simulink model "QDrone_YOLO_Stage6_RealYOLO_MonitorOnly"  (R2021b)
settings: Solver=ode2  StartTime=0.0  StopTime=inf  FixedStep=0.001  RelTol=1e-3  EnableMultiTasking=on
undefined symbols (not defined in the file): Host, qc_get_step_size
libraries: quarc_library x33, simulink x5
(part 2 of 2)

== system QDrone_YOLO_Stage6_RealYOLO_MonitorOnly/MISSION SERVER - LEADER//FOLLOWER with QBot 2e and QDrone/JOYSTICK/Pulse Check ==
  note: For this subsystem we will count the number of new pulses. The data can be considered enabled once the count of new signals has gone beyond 1. This will enable the Initializing and conditioning subsystem.
  new : Inport
  Compare : quarc_library/Logic Operations/Compare  operator=>=  output_data_type=boolean
      settings: SourceProductName=QUARC Targets
  Pulse Check : Constant
  "pulse count " : Subsystem  TreatAsAtomicUnit=on
  signal enable : Outport  InitialOutput=0  VectorParamsAs1DForOutWhenUnconnected=off
  wires:
  Compare/1 -> signal enable/1
  Pulse Check/1 -> Compare/2
  new/1 -> "pulse count "/Trigger
  "pulse count "/1(Number of Pulses) -> Compare/1

== system QDrone_YOLO_Stage6_RealYOLO_MonitorOnly/MISSION SERVER - LEADER//FOLLOWER with QBot 2e and QDrone/Data Server (Localization) /Convention Correction (Motive Frame to Research Studio Frame) - QBot 2e/Prevent Gimbal Lock ==
  note: Remapping the rotation order to prevent gimbal lock
      | in heading/yaw due to Euler singularity condition
  Attitude (rad) [3] : Inport
  Demux : Demux  Outputs=3
  Euler Angles from Rotation Matrix (Relative ZYX) : quarc_library/Math Operations/Matrices/Euler Angles from Rotation Matrix  menu_order=Relative Z-Y-X
      settings: SourceProductName=QUARC Targets
  Euler Angles to Rotation Matrix (Relative YZX) : quarc_library/Math Operations/Matrices/Euler Angles to Rotation Matrix  menu_order=Relative Y-Z-X
      settings: SourceProductName=QUARC Targets
  Mux : Mux  Inputs=3
  "Attitude (rad) [3] " : Outport  VectorParamsAs1DForOutWhenUnconnected=off
  wires:
  Euler Angles from Rotation Matrix (Relative ZYX)/2 -> Mux/2
  Euler Angles from Rotation Matrix (Relative ZYX)/1 -> Mux/3
  Euler Angles from Rotation Matrix (Relative ZYX)/3 -> Mux/1
  Euler Angles to Rotation Matrix (Relative YZX)/1 -> Euler Angles from Rotation Matrix (Relative ZYX)/1
  Attitude (rad) [3]/1 -> Demux/1
  Mux/1 -> "Attitude (rad) [3] "/1
  Demux/2 -> Euler Angles to Rotation Matrix (Relative YZX)/1
  Demux/3 -> Euler Angles to Rotation Matrix (Relative YZX)/2
  Demux/1 -> Euler Angles to Rotation Matrix (Relative YZX)/3

== system QDrone_YOLO_Stage6_RealYOLO_MonitorOnly/MISSION SERVER - LEADER//FOLLOWER with QBot 2e and QDrone/Data Server (Localization) /Convention Correction (Motive Frame to Research Studio Frame) - QDrone/Prevent Gimbal Lock ==
  note: Remapping the rotation order to prevent gimbal lock
      | in heading/yaw due to Euler singularity condition
  Attitude (rad) [3] : Inport
  Demux : Demux  Outputs=3
  Euler Angles from Rotation Matrix (Relative ZYX) : quarc_library/Math Operations/Matrices/Euler Angles from Rotation Matrix  menu_order=Relative Z-Y-X
      settings: SourceProductName=QUARC Targets
  Euler Angles to Rotation Matrix (Relative YZX) : quarc_library/Math Operations/Matrices/Euler Angles to Rotation Matrix  menu_order=Relative Y-Z-X
      settings: SourceProductName=QUARC Targets
  Mux : Mux  Inputs=3
  "Attitude (rad) [3] " : Outport  VectorParamsAs1DForOutWhenUnconnected=off
  wires:
  Euler Angles from Rotation Matrix (Relative ZYX)/2 -> Mux/2
  Euler Angles from Rotation Matrix (Relative ZYX)/1 -> Mux/3
  Euler Angles from Rotation Matrix (Relative ZYX)/3 -> Mux/1
  Euler Angles to Rotation Matrix (Relative YZX)/1 -> Euler Angles from Rotation Matrix (Relative ZYX)/1
  Attitude (rad) [3]/1 -> Demux/1
  Mux/1 -> "Attitude (rad) [3] "/1
  Demux/2 -> Euler Angles to Rotation Matrix (Relative YZX)/1
  Demux/3 -> Euler Angles to Rotation Matrix (Relative YZX)/2
  Demux/1 -> Euler Angles to Rotation Matrix (Relative YZX)/3

== system QDrone_YOLO_Stage6_RealYOLO_MonitorOnly/MISSION SERVER - LEADER//FOLLOWER with QBot 2e and QDrone/JOYSTICK/Pulse Check/pulse count  ==
  Trigger : TriggerPort  TriggerType=either  VariantControl=Variant
  Constant1 : Constant  Value=0
  Increment Stored Integer : simulink/Additional Math & Discrete/Additional Math: Increment - Decrement/Increment Stored Integer
  Sum : Sum  Inputs=|++
  Unit Delay : UnitDelay  SampleTime=-1  HasFrameUpgradeWarning=on
  Number of Pulses : Outport  VectorParamsAs1DForOutWhenUnconnected=off
  wires:
  Constant1/1 -> Sum/1
  Sum/1 -> Increment Stored Integer/1
  Unit Delay/1 -> Sum/2
  Increment Stored Integer/1 -> Unit Delay/1, Number of Pulses/1

== matlab function QDrone_YOLO_Stage6_RealYOLO_MonitorOnly/MISSION SERVER - LEADER//FOLLOWER with QBot 2e and QDrone/Extract Vehicle Data - QBot 2e/Extract Object Data ==
  data: data input; position output; orientation output; index input; tracking output
function [position, orientation, tracking] = fcn(data, index)

n = length(data)/7;

if (index<=0)||(index>n)
    position = zeros(1,3); orientation = zeros(1,3); tracking = 0;
else
    position = [data(index*3-2), data(index*3-1), data(index*3)];
    orientation = [data((index+n)*3 - 2), data((index+n)*3 - 1), data((index+n)*3)];
    tracking = data(index + (n*6));
end

== matlab function QDrone_YOLO_Stage6_RealYOLO_MonitorOnly/MISSION SERVER - LEADER//FOLLOWER with QBot 2e and QDrone/Extract Vehicle Data - QDrone/Extract Object Data ==
  data: data input; position output; orientation output; index input; tracking output
function [position, orientation, tracking] = fcn(data, index)

n = length(data)/7;

if (index<=0)||(index>n)
    position = zeros(1,3); orientation = zeros(1,3); tracking = 0;
else
    position = [data(index*3-2), data(index*3-1), data(index*3)];
    orientation = [data((index+n)*3 - 2), data((index+n)*3 - 1), data((index+n)*3)];
    tracking = data(index + (n*6));
end

== matlab function QDrone_YOLO_Stage6_RealYOLO_MonitorOnly/Communication - QDrone/Detect Communication loss/MATLAB Function ==
  data: time input; stream_connection_loss output; state input; error input
function stream_connection_loss  = fcn(time, state, error)

stream_connection_loss = 0;
if time > 1
    if ~((state == 2)&&(error >= 0))
        % stream connection is not established correctly
        stream_connection_loss = 1;
    end
end

== matlab function QDrone_YOLO_Stage6_RealYOLO_MonitorOnly/Communication - QBot 2e/Detect Communication loss/MATLAB Function ==
  data: time input; stream_connection_loss output; state input; error input
function stream_connection_loss  = fcn(time, state, error)

stream_connection_loss = 0;
if time > 1
    if ~((state == 2)&&(error >= 0))
        % stream connection is not established correctly
        stream_connection_loss = 1;
    end
end

== matlab function QDrone_YOLO_Stage6_RealYOLO_MonitorOnly/MISSION SERVER - LEADER//FOLLOWER with QBot 2e and QDrone/YOLOPoseCommandGenerator ==
  data: measured_pose input; cmd_pose output; detected input; error_x input; error_y input; forward_cmd output; right_cmd output; state output
function [cmd_pose, forward_cmd, right_cmd, state] = YOLOPoseCommandGenerator(measured_pose, detected, error_x, error_y)

% measured_pose = [x; y; z; yaw]
% cmd_pose      = [desired_x; desired_y; desired_z; desired_yaw]

persistent smooth_forward smooth_right centered_counter

if isempty(smooth_forward)
    smooth_forward = 0;
    smooth_right = 0;
    centered_counter = 0;
end

% Parameters
deadband_pixels = 40;
alpha = 0.25;

% Maximum normalized command
max_norm_cmd = 1.0;

% Small pose offset limit for safety
max_position_step = 0.05;   % meters

% Landing disabled for this first test
enable_descent = 0;
descent_step = 0.02;        % meters, later only

centered_required = 10;

% Image size
image_center_x = 320;
image_center_y = 240;

% Read measured pose
x = measured_pose(1);
y = measured_pose(2);
z = measured_pose(3);
yaw = measured_pose(4);

raw_forward = 0;
raw_right = 0;
state = 0;

if detected == 1

    x_centered = abs(error_x) <= deadband_pixels;
    y_centered = abs(error_y) <= deadband_pixels;

    if x_centered && y_centered
        centered_counter = centered_counter + 1;
        state = 2;
    else
        centered_counter = 0;
        state = 1;

        % Calibration-confirmed mapping:
        % error_x > 0 means too forward -> move backward
        % error_x < 0 means too backward -> move forward
        if ~x_centered
            raw_forward = -error_x / image_center_x;
        end

        % error_y > 0 means too right -> move left
        % error_y < 0 means too left -> move right
        if ~y_centered
            raw_right = -error_y / image_center_y;
        end

        raw_forward = min(max(raw_forward, -max_norm_cmd), max_norm_cmd);
        raw_right = min(max(raw_right, -max_norm_cmd), max_norm_cmd);
    end

    if centered_counter >= centered_required
        state = 3;
    end

else
    centered_counter = 0;
    state = 0;
    raw_forward = 0;
    raw_right = 0;
end

% Smooth commands
smooth_forward = alpha * raw_forward + (1 - alpha) * smooth_forward;
smooth_right = alpha * raw_right + (1 - alpha) * smooth_right;

if detected == 0
    smooth_forward = 0.7 * smooth_forward;
    smooth_right = 0.7 * smooth_right;
end

% Convert normalized command to small position offset
forward_offset = max_position_step * smooth_forward;
right_offset = max_position_step * smooth_right;

% Body-frame to world-frame conversion using yaw
dx_world = cos(yaw) * forward_offset - sin(yaw) * right_offset;
dy_world = sin(yaw) * forward_offset + cos(yaw) * right_offset;

desired_x = x + dx_world;
desired_y = y + dy_world;
desired_z = z;
desired_yaw = yaw;

% Descent disabled for first test
if enable_descent == 1 && state == 3
    desired_z = z - descent_step;
end

cmd_pose = [desired_x; desired_y; desired_z; desired_yaw];

forward_cmd = smooth_forward;
right_cmd = smooth_right;

end
